simulink model "model8_agente"  (R2024b)
settings: Solver=VariableStepAuto  StartTime=0.0  StopTime=719  RelTol=1e-3
model workspace (MAT data in the model file):
  agentObj = 67
undefined symbols (not defined in the file): bat_deseado, bat_inicial, dia_radiacion, dia_solar, difh, dni, e_inicial, ghi, glb, n_inicial, seed_radiation, seed_solar, seed_x, seed_y, seed_z, selection, sun_vector, viento
libraries: rllib x2, simulink x1
settings Model: Creator=danie  LastModifiedBy=Daniel
settings SolverCC: ZeroCrossAlgorithm=Adaptive
settings DebuggingCC: IgnoredZcDiagnostic=none

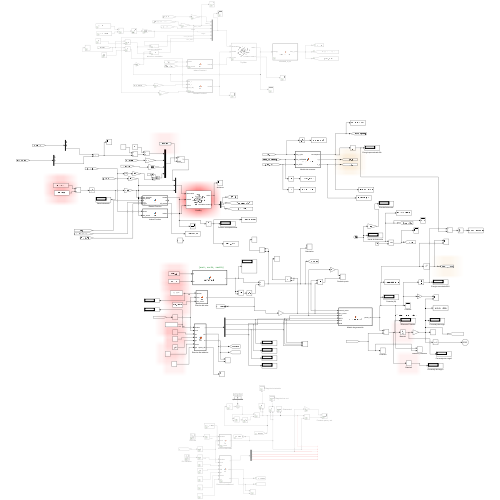
[thumbnail: Simulink's stored preview of the top-level diagram]
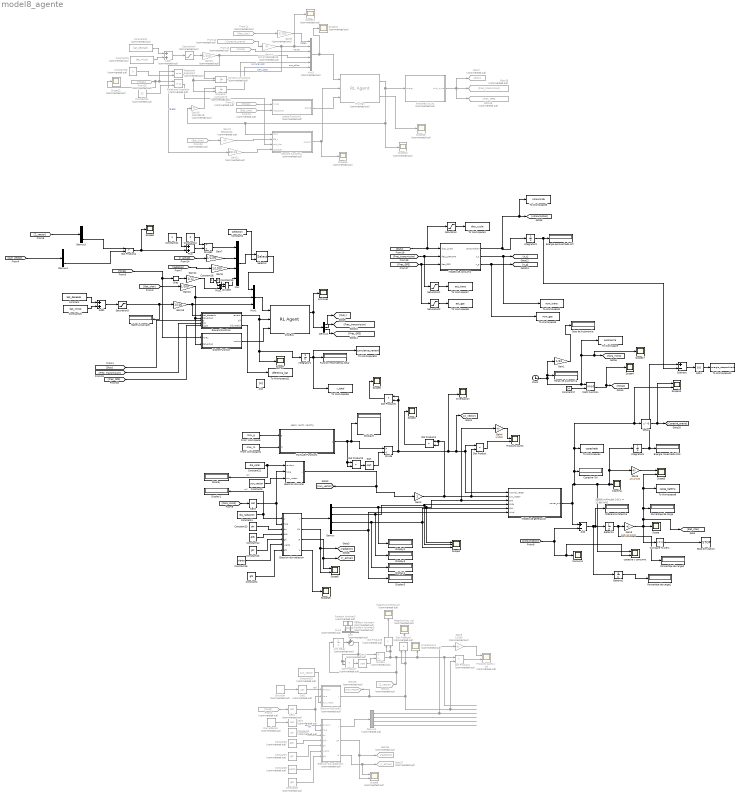
== system model8_agente ==
  note: {east, north, zenith}
  note: $3600\:mAh\cdot 3.6\:V = 12.96\:Wh$
  Abs : Abs  ZeroCross=off  SaturateOnIntegerOverflow=off
  Abs1 : Abs  ZeroCross=off  SaturateOnIntegerOverflow=off
  Acciones : Scope
  Add : Sum  Inputs=+-
  Add1 : Sum
  Add2 : Sum  Commented=on
  Batería buscado : Display
  Batería1 : Integrator  InitialCondition=12.24*2*(bat_inicial/100)  LimitOutput=on  UpperSaturationLimit=12.24*2  LowerSaturationLimit=0  ZeroCross=off
  Batería2 : Integrator  InitialCondition=12.24*2*(bat_inicial/100)  UpperSaturationLimit=12.24*2  LowerSaturationLimit=0
  Bias : Bias  Bias=-12  SaturateOnIntegerOverflow=off
  Ceil1 : Rounding  Commented=on  Operator=ceil
  Ceil2 : Rounding  Commented=on  Operator=ceil
  Ceil3 : Rounding  Operator=ceil
  Ceil4 : Rounding  Commented=on  Operator=ceil
  Clock : Clock
  Compare To Zero : simulink/Logic and Bit Operations/Compare To Zero  relop=<=  OutDataTypeStr=boolean
  Constant : Constant  Value=bat_deseado
  Constant1 : Constant  Value=dia_radiacion
  Constant10 : Constant  Commented=on  Value=sun_vector
  Constant11 : Constant
  Constant12 : Constant  Value=2
  Constant13 : Constant  Value=dni
  Constant14 : Constant  Value=difh
  Constant15 : Constant  Value=ghi
  Constant16 : Constant  Value=viento
  Constant17 : Constant  Value=24
  Constant18 : Constant
  Constant19 : Constant  Value=2
  Constant2 : Constant  Value=glb
  Constant20 : Constant  Value=bat_inicial
  Constant21 : Constant  Value=dia_solar
  Constant22 : Constant  Commented=on  Value=bat_deseado
  Constant23 : Constant  Commented=on  Value=bat_inicial
  Constant24 : Constant  Commented=on  Value=23
  Constant25 : Constant  Commented=on  Value=0
  Constant3 : Constant  Value=sun_vector
  Constant4 : Constant  Value=selection
  Constant5 : Constant  Commented=on  Value=dni
  Constant6 : Constant  Commented=on  Value=difh
  Constant7 : Constant  Commented=on  Value=ghi
  Constant8 : Constant  Commented=on  Value=viento
  Constant9 : Constant  Commented=on  Value=glb
  Consumo : Scope
  Cosecha : Scope
  Cosecha (W) : Display
  CowBoy : rllib/RL Agent  Agent=agent  ExternalActionAsInput=off  ProvideLastAction=off  ProvideCumRwd=on  TreatAsDirectFeedthrough=on  UseStrictObservationDataTypes=off
  Delay : Delay  DelayLength=0  SampleTime=1
  Demux : Demux
  Demux1 : Demux  Outputs=3
  Demux2 : Demux  Commented=on
  Demux3 : Demux  Outputs=3
  Demux4 : Demux  Outputs=3
  Diferencia Potencia : Display
  Display{,1..6} (7 alike) : Display
  Divide : Product  Inputs=*/
  Divide1 : Product  Commented=on  Inputs=*/
  Divide2 : Product  Inputs=/*
  Divide3 : Product  Inputs=/*
  Dot Product{,1,3..5} (5 alike) : DotProduct  OutDataTypeStr=Inherit: Inherit via internal rule
  Dot Product{2,6..8} (4 alike) : DotProduct  Commented=on  OutDataTypeStr=Inherit: Inherit via internal rule
  Día radiacion : UniformRandomNumber  Commented=on  Minimum=1  Maximum=4383  Seed=seed_radiation  SampleTime=24
  Día solar : UniformRandomNumber  Commented=on  Minimum=1  Maximum=365  Seed=seed_solar  SampleTime=24
  Días de Autonomía : Display
  Eleccion día radiacion : MATLAB Function  TreatAsAtomicUnit=on
  Eleccion día radiacion1 : MATLAB Function  Commented=on  TreatAsAtomicUnit=on
  Eleccion día solar : MATLAB Function  TreatAsAtomicUnit=on
  Eleccion día solar1 : MATLAB Function  Commented=on  TreatAsAtomicUnit=on
  Energia aprovechada Wh : Display
      settings: Decimation=5
  Energia cosechada Wh3 : Display
      settings: Decimation=5
  From Workspace : FromWorkspace  VariableName=mov_g  SampleTime=1
  From Workspace1 : FromWorkspace  VariableName=mov_m  SampleTime=1
  From11 : From  Commented=on  GotoTag=Bat_char
  From12 : From  Commented=on  GotoTag=Cosecha_previa
  From{2,13,20,22} (4 alike) : From  Commented=on  GotoTag=horas
  From21 : From  Commented=on  GotoTag=Bat_char
  From23 : From  Commented=on  GotoTag=Bat_char
  Funcion recompensa total : Display
      settings: Decimation=5
  Gain1 : Gain  Gain=1/24
  Gain10 : Gain  Gain=1/100
  Gain11 : Gain  Commented=on  Gain=88128
  Gain12 : Gain  Gain=1/12
  Gain13 : Gain  Gain=1/100
  Gain14 : Gain  Commented=on  Gain=157.5*3600/88128
  Gain15 : Gain  Commented=on  Gain=1/100
  Gain16 : Gain  Commented=on  Gain=100/(88128)
  Gain17 : Gain  Commented=on  Gain=88128/100
  Gain2 : Gain
  Gain3 : Gain  Gain=100/(12.24*2)
  Gain4 : Gain  Gain=1/1000
  Gain5 : Gain  Commented=on  Gain=1/1000
  Gain6 : Gain  Gain=1/0.4*100
  Gain7 : Gain  Gain=1/1200
  Gain8 : Gain  Commented=on  Gain=1/100
  Gain9 : Gain  Gain=1/1200
  Goto14 : Goto  Commented=on  GotoTag=Z_vector
  Goto15 : Goto  Commented=on  GotoTag=sun_vector
  Goto16 : Goto  Commented=on  GotoTag=radiation
  Goto17 : Goto  Commented=on  GotoTag=r_actual
  Goto18 : Goto  Commented=on  GotoTag=Frec_transmision
  Goto19 : Goto  Commented=on  GotoTag=Frec_GPS
  Goto7 : Goto  Commented=on  GotoTag=Duty
  Horas de Autonomía : Display
  Integrator1 : Integrator
  Integrator3 : Integrator
  Integrator6 : Integrator
  Isdone Function : MATLAB Function  TreatAsAtomicUnit=on
  Isdone Function1 : MATLAB Function  Commented=on  TreatAsAtomicUnit=on
  MATLAB Function1 : MATLAB Function  TreatAsAtomicUnit=on
  Magnitud orientación : Scope  Commented=on
  Magnitud vec. sol : Scope  Commented=on
  Math Function : Math  Operator=mod
  Modelo de consumo : MATLAB Function  TreatAsAtomicUnit=on
  Modelo de generación : MATLAB Function  TreatAsAtomicUnit=on
  Mux : Mux
  Mux1 : Mux  Inputs=3
  Mux2 : Mux  Commented=on  Inputs=3
  Mux3 : Mux  Commented=on  Inputs=6
  Orientacion : Scope  NumInputPorts=2
  Orientacion1 : Scope  Commented=on  NumInputPorts=2
  Plus : Sum
  Plus1 : Sum
  Porcentaje de carga : Display
  Porcentaje de carga1 : Display
  Porcentaje de carga2 : Display
  Producto punto : Scope  NumInputPorts=2
  Producto punto y sol : Scope  Commented=on  NumInputPorts=2
  Random Number3 : RandomNumber  Commented=on  Variance=0.05  Seed=seed_x  SampleTime=1
  Random Number4 : RandomNumber  Commented=on  Variance=0.05  Seed=seed_y  SampleTime=1
  Random Number5 : RandomNumber  Commented=on  Variance=0.05  Seed=seed_z  SampleTime=1
  Relational Operator : RelationalOperator  Commented=on  OutDataTypeStr=boolean  ZeroCross=off  RndMeth=Simplest  InputSameDT=off
  Relational Operator1 : RelationalOperator  Commented=on  Operator===  OutDataTypeStr=boolean  ZeroCross=off  RndMeth=Simplest  InputSameDT=off
  Reward Function : MATLAB Function  TreatAsAtomicUnit=on
  Reward Function1 : MATLAB Function  Commented=on  TreatAsAtomicUnit=on
  Saturation : Saturate  UpperLimit=1  LowerLimit=0.1
  Saturation1 : Saturate  UpperLimit=1  LowerLimit=0.1
  Saturation2 : Saturate  UpperLimit=1  LowerLimit=0.1
  Saturation3 : Saturate  UpperLimit=100  LowerLimit=1
  Saturation4 : Saturate  Commented=on  UpperLimit=100  LowerLimit=1
  Scope{,2,4,6..7,9,17..18} (8 alike) : Scope
  Scope1 : Scope  NumInputPorts=3
  Scope{10..13,15..16} (6 alike) : Scope  Commented=on
  Scope14 : Scope  NumInputPorts=2
  Scope3 : Scope  NumInputPorts=2
  Scope5 : Scope  NumInputPorts=2
  Scope8 : Scope  Commented=on  NumInputPorts=2
  Selector : Selector  InputPortWidth=4  IndexOptions=Index vector (port)  Indices=[1 3]  OutputSizes=1
  Sqrt : Sqrt
  Sqrt1 : Sqrt  Commented=on
  Stop Simulation : Stop
  Subtract : Sum  Inputs=+-
  Sum : Sum  Commented=on  Inputs=++|
  TinyMan : rllib/RL Agent  Commented=on  Agent=agent  ExternalActionAsInput=off  ProvideLastAction=off  ProvideCumRwd=on  TreatAsDirectFeedthrough=on  UseStrictObservationDataTypes=off
  To Workspace : ToWorkspace  VariableName=autonomia  SaveFormat=Timeseries  SampleTime=1
  To Workspace1 : ToWorkspace  VariableName=duty_cycle  SaveFormat=Timeseries  SampleTime=1
  To Workspace10 : ToWorkspace  VariableName=cumulative_reward  SaveFormat=Timeseries  SampleTime=1
  To Workspace11 : ToWorkspace  VariableName=diferencia_bat  SaveFormat=Timeseries  SampleTime=1
  To Workspace12 : ToWorkspace  VariableName=energia_desperdiciada  SaveFormat=Timeseries  SampleTime=1
  To Workspace2 : ToWorkspace  VariableName=num_trans  SaveFormat=Timeseries  SampleTime=1
  To Workspace3 : ToWorkspace  VariableName=num_gps  SaveFormat=Timeseries  SampleTime=1
  To Workspace4 : ToWorkspace  VariableName=cosechada  SaveFormat=Timeseries  SampleTime=1
  To Workspace5 : ToWorkspace  VariableName=consumida  SaveFormat=Timeseries  SampleTime=1
  To Workspace6 : ToWorkspace  VariableName=carga_bateria  SaveFormat=Timeseries  SampleTime=1
  To Workspace7 : ToWorkspace  VariableName=act_trans  SaveFormat=Timeseries  SampleTime=-1
  To Workspace8 : ToWorkspace  VariableName=act_gps  SaveFormat=Timeseries  SampleTime=-1
  To Workspace9 : ToWorkspace  VariableName=r_total  SaveFormat=Timeseries  SampleTime=1
  Unit Delay : UnitDelay  Commented=on  InitialCondition=[e_inicial n_inicial 1]  HasFrameUpgradeWarning=on
  allocated_to_dc : MATLAB Function  Commented=on  TreatAsAtomicUnit=on
  allocation cumulative : Integrator  Commented=on  ExternalReset=rising  UpperSaturationLimit=12.24*2  LowerSaturationLimit=0
  cosecha y consumo : Scope  NumInputPorts=2
  harvest cumulative : Integrator  Commented=on  ExternalReset=rising  UpperSaturationLimit=12.24*2  LowerSaturationLimit=0
  wires:
  Clock/1 -> To Workspace/1, Scope17/1, [hora_inicio], Math Function/1, Gain1/1, Horas de Autonomía/1
  Gain1/1 -> Días de Autonomía/1
  Demux/2 -> Display3/1, Modelo de generación/4(DIFH), Scope1/2
  Demux/3 -> Display4/1, Modelo de generación/5(GHI), Scope1/3
  Demux/4 -> Modelo de generación/6(wind), Display5/1
  Gain2/1 -> Dot Product1/2, Dot Product1/1, Modelo de generación/2(sun_vector), Dot Product/2
  Dot Product/1 -> Producto punto/2
  Dot Product1/1 -> Scope2/1
  Eleccion día solar/1(y) -> Gain2/1, [sun_vector]
  Gain4/1 -> Producto punto/1
  Dot Product3/1 -> Sqrt/1
  Eleccion día radiacion/1(y) -> Demux/1
  Ceil3/1 -> Eleccion día radiacion/2(hora), Eleccion día solar/2(hora)
  Constant21/1 -> Display/1, Eleccion día solar/1(random)  "roll"
  Constant13/1 -> Eleccion día radiacion/3(dni)
  Constant14/1 -> Eleccion día radiacion/4(difh)
  Constant15/1 -> Eleccion día radiacion/5(ghi)
  Constant16/1 -> Eleccion día radiacion/6(viento)
  Constant3/1 -> Eleccion día solar/3(sun_vector)
  [hora_inicio] -> Ceil3/1
  Eleccion día radiacion/2(r24) -> [radiation], Scope5/2
  Math Function/1 -> Scope4/1, [horas]
  Constant17/1 -> Math Function/2
  Sqrt/1 -> Divide/2
  Dot Product5/1 -> Scope6/1
  Divide/1 -> Orientacion/2, [Z_vector], Modelo de generación/1(normal_vector), Dot Product/1, Dot Product5/1, Dot Product5/2
  [Frec_transmision] -> Modelo de consumo/2(frec_LoRAWAN), Saturation1/1
  [Frec_GPS] -> Modelo de consumo/3(frec_GPS), Saturation2/1
  Modelo de consumo/2(n_t) -> To Workspace2/1, [n_t]
  Modelo de consumo/3(n_g) -> To Workspace3/1, [n_g]
  Demux/1 -> Display2/1, Scope1/1, Modelo de generación/3(DNI), Gain4/1
  Constant2/1 -> Eleccion día radiacion/7(glb)
  From Workspace/1 -> MATLAB Function1/1(g)
  From Workspace1/1 -> MATLAB Function1/2(m)
  MATLAB Function1/1(z) -> Dot Product3/2, Dot Product3/1, Display6/1, Divide/1
  Constant1/1 -> Display1/1, Eleccion día radiacion/1(random)  "roll"
  Saturation/1 -> To Workspace1/1
  Saturation1/1 -> To Workspace7/1
  Saturation2/1 -> To Workspace8/1
  Gain9/1 -> Mux/3
  Mux/1 -> Selector/1
  Gain13/1 -> Mux1/3, Reward Function/1(bat_deseado)
  Constant20/1 -> Add1/2
  Demux3/3 -> Dot Product4/1
  Gain12/1 -> Plus1/2
  [Frec_transmision] -> Reward Function/4(f_tx)
  Selector/1 -> Mux1/1
  [horas] -> Isdone Function/1(horas), Bias/1
  Bias/1 -> Gain12/1
  Gain7/1 -> Mux/2
  [radiation] -> Gain9/1
  Demux1/3 -> [Frec_GPS]
  Constant/1 -> Add1/1
  CowBoy/1 -> Demux1/1, Acciones/1
  Mux1/1 -> CowBoy/1
  Add1/1 -> Saturation3/1
  Demux1/2 -> [Frec_transmision]
  Gain10/1 -> Isdone Function/2(bat_actual), Reward Function/2(bat_actual), Mux1/2
  Reward Function/1(reward) -> Integrator1/1, Scope7/1, CowBoy/2
  Demux1/1 -> [Duty]
  [Frec_GPS] -> Reward Function/5(f_gps)
  [r_actual] -> Gain7/1
  [Bat_char] -> Gain10/1
  Constant4/1 -> Selector/2
  Dot Product4/1 -> Scope9/1, Plus/2
  Isdone Function/1(isdone) -> CowBoy/3
  [sun_vector] -> Demux4/1
  Demux2/3 -> ?
  Demux2/2 -> ?
  Ceil2/1 -> Eleccion día radiacion1/1(random)  "roll"
  Unit Delay/1 -> Sum/2
  Mux2/1 -> Sum/1
  Random Number4/1 -> Mux2/2
  Eleccion día solar1/1(y) -> Dot Product2/2, Dot Product6/1, Dot Product6/2, Goto15/1
  Día radiacion/1 -> Ceil2/1
  Sum/1 -> Dot Product7/2, Dot Product7/1, Divide1/1
  Constant10/1 -> Eleccion día solar1/3(sun_vector)
  Divide1/1 -> Unit Delay/1, Goto14/1, Dot Product2/1, Orientacion1/2, Dot Product8/1, Dot Product8/2
  Eleccion día radiacion1/2(r24) -> Goto16/1, Scope8/2
  Dot Product8/1 -> Magnitud orientación/1
  Demux2/1 -> Gain5/1
  Ceil1/1 -> Eleccion día solar1/1(random)  "roll"
  Eleccion día radiacion1/1(y) -> Demux2/1
  Random Number3/1 -> Mux2/1
  Constant6/1 -> Eleccion día radiacion1/4(difh)
  Constant9/1 -> Eleccion día radiacion1/7(glb)
  Constant8/1 -> Eleccion día radiacion1/6(viento)
  Eleccion día radiacion1/3(ra) -> Scope8/1, Goto17/1
  Dot Product7/1 -> Sqrt1/1
  Constant5/1 -> Eleccion día radiacion1/3(dni)
  Constant7/1 -> Eleccion día radiacion1/5(ghi)
  Día solar/1 -> Ceil1/1
  Gain5/1 -> Producto punto y sol/1
  Random Number5/1 -> Mux2/3
  Sqrt1/1 -> Divide1/2
  Dot Product6/1 -> Magnitud vec. sol/1
  Demux2/4 -> ?
  From2/1 -> Ceil4/1
  Dot Product2/1 -> Producto punto y sol/2
  Ceil4/1 -> Eleccion día radiacion1/2(hora), Eleccion día solar1/2(hora)
  Gain6/1 -> Scope3/1
  [consumption] -> cosecha y consumo/2, Consumo/1, Add/2
  Gain3/1 -> Compare To Zero/1, [Bat_char], To Workspace6/1, Scope3/2, Porcentaje de carga/1, Scope/1
  Batería1/1 -> Porcentaje de carga2/1, Gain3/1
  Add/1 -> Batería2/1, Batería1/1, Diferencia Potencia/1
  Compare To Zero/1 -> Stop Simulation/1
  Plus/1 -> Divide2/2
  Constant11/1 -> Plus/1
  Constant12/1 -> Divide2/1
  Divide2/1 -> Mux/1
  Constant19/1 -> Divide3/1
  Constant18/1 -> Plus1/1
  Plus1/1 -> Divide3/2
  Divide3/1 -> Mux/4
  Saturation3/1 -> Batería buscado/1, Gain13/1
  [Duty] -> Reward Function/3(D)
  [Z_vector] -> Demux3/1
  Demux4/3 -> Dot Product4/2
  Integrator1/1 -> To Workspace9/1, To Workspace10/1, Funcion recompensa total/1
  Reward Function/3(dif_notabs) -> To Workspace11/1
  Integrator6/1 -> Subtract/1, Energia cosechada Wh3/1
  Integrator3/1 -> Subtract/2, Energia aprovechada Wh/1
  Subtract/1 -> Abs1/1
  [Duty] -> Saturation/1, Modelo de consumo/1(duty_cycle)
  Modelo de consumo/1(consumption) -> To Workspace5/1, [consumption], Integrator3/1
  Abs1/1 -> To Workspace12/1
  Constant24/1 -> Relational Operator/2
  TinyMan/1 -> Scope10/1, Reward Function1/1(EA_t), Gain16/1, allocated_to_dc/1(energy)
  From22/1 -> Isdone Function1/1(horas)
  Gain17/1 -> Reward Function1/2(EB_t)
  Gain8/1 -> Mux3/1  "batery"
  Constant23/1 -> Add2/2
  harvest cumulative/1 -> Mux3/5  "cum_harvest"
  Isdone Function1/1(isdone) -> TinyMan/3
  allocated_to_dc/1(duty_cycle) -> Goto19/1, Goto7/1, Goto18/1
  From12/1 -> Gain14/1
  Relational Operator/1 -> Reward Function1/3(end_day)
  Gain14/1 -> harvest cumulative/1, Scope13/1, Mux3/2  "prev_cose"
  From23/1 -> Gain17/1
  Constant22/1 -> Add2/1
  Gain15/1 -> Gain11/1, Mux3/4  "target"
  Gain11/1 -> Reward Function1/4(E_target)
  From11/1 -> Gain8/1
  Saturation4/1 -> Gain15/1
  From21/1 -> Isdone Function1/2(bat_actual)
  Add2/1 -> Saturation4/1
  Mux3/1 -> Scope11/1, TinyMan/1
  From13/1 -> Mux3/3  "houra"
  allocation cumulative/1 -> Mux3/6  "cum_alloc"
  Reward Function1/1(reward) -> Scope15/1, TinyMan/2
  From20/1 -> Scope12/1, Relational Operator1/1, Relational Operator/1
  Gain16/1 -> allocation cumulative/1
  Constant25/1 -> Relational Operator1/2
  Relational Operator1/1 -> allocation cumulative/2, harvest cumulative/2
  Modelo de generación/1(power_out) -> cosecha y consumo/1, Integrator6/1, Gain6/1, Cosecha/1, Scope14/2, Delay/1, To Workspace4/1, Cosecha (W)/1, Add/1
  Delay/1 -> Scope14/1, [Cosecha_previa]
  TinyMan/2 -> Scope16/1
  Batería2/1 -> Porcentaje de carga1/1
  Eleccion día radiacion/3(ra) -> Scope5/1, [r_actual]
  Eleccion día radiacion/4(ajuste_dia) -> Scope18/1

== matlab function model8_agente/Modelo de generación ==
  data: normal_vector input; power_out output; sun_vector input; DNI input; DIFH input; GHI input; wind input
function power_out  = radiation_model(normal_vector,sun_vector,DNI,DIFH,GHI,wind)

%   By: Daniel Iglesias - UFRO - 2024

%   Modelo basado en "Modelo de Generación Fotovoltaica" de Alejandra
%   Molina Monje y Francisco martínez (Marzo 2017)
%   Disponible en: https://solar.minenergia.cl/downloads/fotovoltaico.pdf
%   [Consultado el 25-11-2024]

% Normal vector:
% Vector normal al panel solar, en formato:
% [Este, Norte, Zenith]
% 
% Sun vector:
% Vector de posición del sol, en formato:
% [Este, Norte, Zenith]

%% Parametros
efficiency = 0.34;
panel_power = 0.3; % Potencia nominal de la instalación
coef_temp = -0.002; % Coeficiencte de temperatura de la celda para su potencia máxima
I_o = 1000; % Radiación de referencia
T_o = 25; % Temperatura de referencia
dT = -0.0471;
a = -2.98;
b = -0.0471;
albedo = 0.24;

%% Módulo de Radiación

% Radiación directa:
dir_inc = max(0,DNI*dot(normal_vector,sun_vector));

% Radiación difusa del cielo
dif_inc = DIFH*0.5*(1 + dot(normal_vector,[0 0 1]));

% Radiación difusa del suelo
dif_suelo = GHI*0.5*albedo*(1 + dot(normal_vector,[0 0 1]));

% Radiación total que incide en un plano inclinado:
incident_rad = dir_inc + dif_inc + dif_suelo;

%% Módulo de reflexión

% El panel utilizado no presenta una cubierta, por lo que no se consideró
% el uso de este módulo.


%% Módulo de Temperatura

% Temperatura de celda:

T_c = dT*incident_rad/1000 + incident_rad*exp(a + b*wind);

%% Módulo de Operación

% Potencia generada
high_power = incident_rad/I_o*panel_power*(1 + coef_temp*(T_c-T_o));
low_power = 0.008*incident_rad^2/I_o * panel_power*(1 + coef_temp*(T_c-T_o));

if incident_rad >= 125
    power_generated = high_power;
else
    power_generated = low_power;
end

%% Módulo de Inversor & Módulo de Pérdidas

%power_out = efficiency*power_generated;
power_out = 1.4327*power_generated^3 - 1.5697*power_generated^2 + 0.6165*power_generated - 0.0005;

end

% glb [W/m2]: Radiación Global
% dir [W/m2]: Radiación Directa
% dif [W/m2]: Radiación Difusa
% sct [W/m2]: Radiación Difusa Relejada
% ghi [W/m2]: Radiación Global Horizontal
% dirh [W/m2]: Radiación Directa
% difh [W/m2]: Radiación Difusa
% dni [W/m2]: Radiación Directa Normal
% temp [C]: Temperatura en 2 metros (correjida)
% vel [m/s]: Velocidad de Viento
% shadow [0: sin, 1: con]: Sobra debido a topografía
% cloud [1: si, 0: no]: Presencia de nubes

== matlab function model8_agente/Isdone Function1 ==
  data: horas input; isdone output; bat_actual input
function isdone = fcn(horas,bat_actual)

    %isdone = (horas==24)||(bat_actual<=0);
    isdone = (horas==24);

== matlab function model8_agente/Reward Function1 ==
  data: EA_t input; reward output; EB_t input; end_day input; E_target input
function reward = fcn(EA_t,EB_t,end_day,E_target)

reward = 0;

if end_day == false
    if EB_t >= 88128/100
        reward = log(EA_t/16.326);
    elseif EB_t < 88128/100 && EB_t > 0
        reward = -abs(EB_t-88128/100)/612;
    else
        reward = -abs(EB_t-E_target)/612;
    end

else 
    reward = -5*abs(EB_t-E_target)/612;
end

== matlab function model8_agente/allocated_to_dc ==
  data: energy input; duty_cycle output
function duty_cycle  = allocated_to_dc(energy)

duty_cycle = energy/112.715;

if (duty_cycle < 0.1)
    duty_cycle = 0.1;
end

if (duty_cycle > 1)
    duty_cycle = 1;
end

end

== matlab function model8_agente/Modelo de consumo ==
  data: duty_cycle input; consumption output; frec_LoRAWAN input; frec_GPS input; n_t output; n_g output
function [consumption, n_t, n_g] = consume_model(duty_cycle, frec_LoRAWAN, frec_GPS)

%% Parametros
modo_activo = 0.095; % CPU
modo_lightsleep = 0.000792; % ULP
modo_deepsleep = 0.0000264; % Sleep

processing_time = 2/3600;

consumo_WT = 0.0000231;

icm42670_activo = 0.001814;
icm42670_sleep = 0.00001155;

transmision_power = 0.254;
transmision_time = 1.133/3600;

GPS_power = 0.437;
GPS_time = 48.520/3600;

%% Parametros JouleScope

modo_activo = 0; % CPU
modo_lightsleep = 0; % ULP
modo_deepsleep = 0; % Sleep

processing_time = 0;

consumo_WT = 0;

icm42670_activo = 0.00872307;
icm42670_sleep = 0.00156235;

%transmision_power = 0.17865;
transmision_power = 0.366;
transmision_time = 10.31/3600;

GPS_power = 0.49475;
GPS_time = 8.81/3600;

%% Ecuacion consumo

modo_activo_time = (duty_cycle*3600/10)*processing_time;
modo_deepsleep_time = 1 - modo_activo_time;

consumo_sensor = duty_cycle*icm42670_activo + (1-duty_cycle)*icm42670_sleep + modo_activo_time*modo_activo + modo_deepsleep_time*modo_deepsleep + consumo_WT;

%% MODIFICADO PARA MAXIMO 20

if frec_LoRAWAN >= 1
    n_t = 10;
elseif frec_LoRAWAN >= 0.1
    n_t = fix(frec_LoRAWAN*10);
else
    n_t = 1;
end

if frec_GPS >= 1
    n_g = 10;
elseif frec_GPS >= 0.1
    n_g = fix(frec_GPS*10);
else
    n_g = 1;
end


consumo_gps = transmision_power*transmision_time*n_t;

consumo_transmision = GPS_power*GPS_time*n_g;

consumption = consumo_sensor + consumo_gps + consumo_transmision;

end

== matlab function model8_agente/Eleccion día solar ==
  data: random input; y output; hora input; sun_vector input
function y = fcn(random,hora,sun_vector)

y = zeros(3, 1);
hora = fix(hora);

n_inicial = (random-1)*24 + 1;

if n_inicial+hora > 8761
    corr_hora = -8761;
else
    corr_hora = 0;
end

y(1) = sun_vector(n_inicial+hora+corr_hora,1);
y(2) = sun_vector(n_inicial+hora+corr_hora,2);
y(3) = sun_vector(n_inicial+hora+corr_hora,3);

== matlab function model8_agente/Eleccion día radiacion ==
  data: random input; y output; hora input; dni input; difh input; ghi input; viento input; r24 output; ra output; glb input; ajuste_dia output
function [y,r24,ra,ajuste_dia] = fcn(random,hora,dni,difh,ghi,viento,glb)

y = zeros(4, 1);
hora = fix(hora);
%r24 = zeros(24,1);

r24 = 0;

n_inicial = (random - 1)*24 + 1;
%n_final = n_inicial+24;

if n_inicial+hora >= 113857
    corr_hora = -364*24;
else
    corr_hora = 0;
end

y(1) = dni(n_inicial+hora+corr_hora,2);
y(2) = difh(n_inicial+hora+corr_hora,2);
y(3) = ghi(n_inicial+hora+corr_hora,2);
y(4) = viento(n_inicial+hora+corr_hora,2);
ra = glb(n_inicial+hora+corr_hora,2);


ajuste_dia = fix(hora/24)*24;

for k = 0:23
    r24 = r24 + glb(n_inicial+k+corr_hora+ajuste_dia,2) + 100;
end

r24 = r24/24;


% y(1) = dni;
% y(2) = difh;
% y(3) = ghi;
% y(4) = viento;

== matlab function model8_agente/Reward Function ==
  data: bat_deseado input; reward output; bat_actual input; D input; f_tx input; f_gps input; dif output; dif_notabs output
function [reward,dif,dif_notabs]= fcn(bat_deseado,bat_actual,D,f_tx,f_gps)

dif = abs(bat_deseado-bat_actual);
dif_notabs = bat_deseado-bat_actual;

% reward = 0.5*(dif<=0.02) - 0.05*dif - 10*(bat_actual<=0);

a=0.5;
b=0.5;
c=0.5;
d=500;
e=10;

% a=10;
% b=0.25;
% c=0.25;
% d=500;
% e=10;

reward = a*D+b*f_tx+c*f_gps-d*dif-e*(bat_actual<=0);

== matlab function model8_agente/Isdone Function ==
  data: horas input; isdone output; bat_actual input
function isdone = fcn(horas,bat_actual)

    isdone = (horas==24)||(bat_actual<=0);

== matlab function model8_agente/Eleccion día radiacion1 ==
  data: random input; y output; hora input; dni input; difh input; ghi input; viento input; r24 output; ra output; glb input
function [y,r24,ra] = fcn(random,hora,dni,difh,ghi,viento,glb)

y = zeros(4, 1);
hora = fix(hora);
%r24 = zeros(24,1);

r24 = 0;

n_inicial = (random - 1)*24 + 1;
%n_final = n_inicial+24;

y(1) = dni(n_inicial+hora,2);
y(2) = difh(n_inicial+hora,2);
y(3) = ghi(n_inicial+hora,2);
y(4) = viento(n_inicial+hora,2);
ra = glb(n_inicial+hora,2);

for k = 0:23
    r24 = r24 + glb(n_inicial+k,2);
end

r24 = r24/24;


% y(1) = dni;
% y(2) = difh;
% y(3) = ghi;
% y(4) = viento;

== matlab function model8_agente/MATLAB Function1 ==
  data: g input; z output; m input
function z = normal_vector(g,m)
%NORMAL_VECTOR Summary of this function goes here
% Por Daniel Iglesias 2024

%{x y z}
% g = [gx gy gz];
% m = [mx my mz];

%magnitud de los vectores
m_m = (m(1)^2+m(2)^2+m(3)^2)^(1/2);
m_g = (g(1)^2+g(2)^2+g(3)^2)^(1/2);

%coeficientes
A = m(1)/m_m;
B = m(2)/m_m;
C = m(3)/m_m;
D = -g(1)/m_g;
E = -g(2)/m_g;
F = -g(3)/m_g;
G = (m(3)*g(2)-m(2)*g(3))/(m_g*m_m);
H = (m(1)*g(3)-m(3)*g(1))/(m_g*m_m);
I = (m(2)*g(1)-m(1)*g(2))/(m_g*m_m);

div = (A*E*I+B*F*G+C*D*H)-(G*E*C+H*F*A+I*D*B);

% vector normal {east, north, zenith}
z = [(A*E-D*B), (D*H-G*E), (B*G-H*A)]/div;

% opuesto al vector normal
%z_p = -z

end

== matlab function model8_agente/Eleccion día solar1 ==
  data: random input; y output; hora input; sun_vector input
function y = fcn(random,hora,sun_vector)

y = zeros(3, 1);
hora = fix(hora);

n_inicial = (random-1)*24 + 1;

y(1) = sun_vector(n_inicial+hora,1);
y(2) = sun_vector(n_inicial+hora,2);
y(3) = sun_vector(n_inicial+hora,3);
